simulink library "ConverterLibrary"  (R2026a)
settings: Solver=VariableStepAuto
undefined symbols (not defined in the file or in its folder): DiscIntNeverNeededParam, dspblkCoreblockFVToolHelper, gcbh, gridInverter
libraries: fl_lib x240, nesl_utility x221, ee_lib x208, slpidlib x28, eeGeneralControl x12, simulink x9, eeTransforms x4, simulink_extras x1, eePowerMeasurement x1
(part 7 of 30)

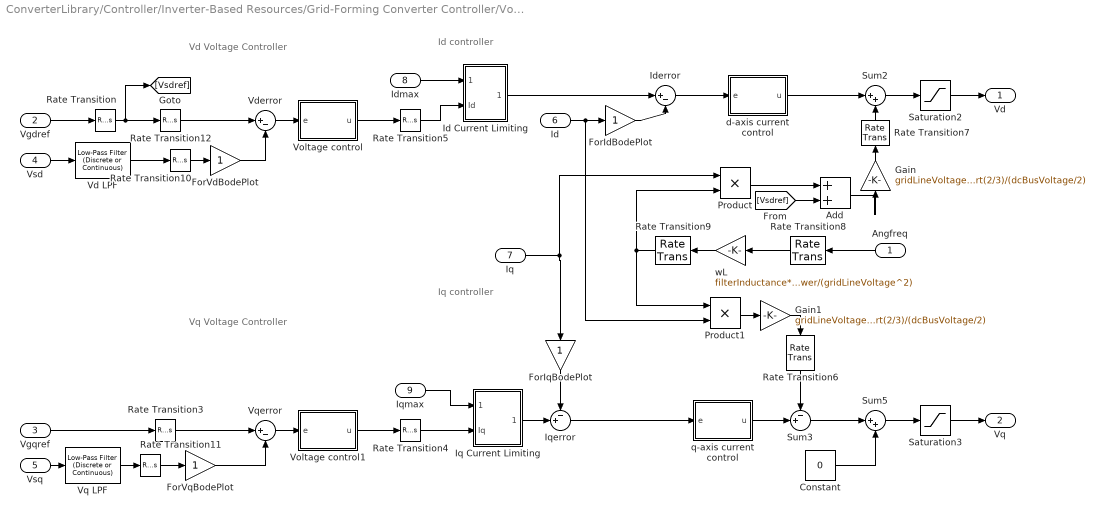
== system ConverterLibrary/Controller/Inverter-Based Resources/Grid-Forming Converter Controller/VoltageCurrentControl/Controller ==
  note: Vq Voltage Controller
  note: Iq controller
  note: Vd Voltage Controller
  note: Id controller
  Angfreq : Inport
  Vgdref : Inport  Port=2
  Vgqref : Inport  Port=3
  Vsd : Inport  Port=4
  Vsq : Inport  Port=5
  Id : Inport  Port=6
  Iq : Inport  Port=7
  Idmax : Inport  Port=8
  Iqmax : Inport  Port=9
  Add : Sum
  Constant : Constant  Value=0  SampleTime=currentControlTs
  ForIdBodePlot : Gain
  ForIqBodePlot : Gain
  ForVdBodePlot : Gain
  ForVqBodePlot : Gain
  Gain : Gain  Gain=gridLineVoltage*sqrt(2/3)/(dcBusVoltage/2)
  Gain1 : Gain  Gain=gridLineVoltage*sqrt(2/3)/(dcBusVoltage/2)
  Id Current Limiting : Subsystem
  Iderror : Sum  Inputs=|+-
  Iq Current Limiting : Subsystem
  Iqerror : Sum  Inputs=-+|
  Product : Product
  Product1 : Product
  Rate Transition{,3..12} (11 alike) : RateTransition
  Saturation2 : Saturate  UpperLimit=4  LowerLimit=-3
  Saturation3 : Saturate  UpperLimit=3  LowerLimit=-3
  Sum2 : Sum  Inputs=|++
  Sum3 : Sum  Inputs=-+|
  Sum5 : Sum  Inputs=|++
  Vd LPF : eeGeneralControl/Low-Pass Filter (Discrete or Continuous)  K=1  T=vdvqLPFTimeConst  B=inf  A=-inf  init_option=Specify as parameter  x0=0  Ts=voltControlTs
  Vderror : Sum  Inputs=|+-
  Voltage control : Subsystem
  Voltage control1 : Subsystem
  Vq LPF : eeGeneralControl/Low-Pass Filter (Discrete or Continuous)  K=1  T=vdvqLPFTimeConst  B=inf  A=-inf  init_option=Inherited from block input  x0=0  Ts=voltControlTs
  Vqerror : Sum  Inputs=|+-
  d-axis current control : Subsystem
  q-axis current control : Subsystem
  wL : Gain  Gain=filterInductance*power/(gridLineVoltage^2)
  Vd : Outport  VectorParamsAs1DForOutWhenUnconnected=off
  Vq : Outport  Port=2  VectorParamsAs1DForOutWhenUnconnected=off
  wires:
  Rate Transition12/1 -> Vderror/1
  Rate Transition11/1 -> ForVqBodePlot/1
  Rate Transition10/1 -> ForVdBodePlot/1
  Vd LPF/1 -> Rate Transition10/1
  ForVqBodePlot/1 -> Vqerror/2
  ForVdBodePlot/1 -> Vderror/2
  Rate Transition9/1 -> Product1/1, Product/2
  Vq LPF/1 -> Rate Transition11/1
  Rate Transition8/1 -> wL/1
  Rate Transition7/1 -> Sum2/2
  Rate Transition6/1 -> Sum3/1
  Rate Transition5/1 -> Id Current Limiting/2(Id)
  Rate Transition4/1 -> Iq Current Limiting/2(Iq)
  Rate Transition3/1 -> Vqerror/1
  Rate Transition/1 -> Rate Transition12/1, [Vsdref]
  Vgdref/1 -> Rate Transition/1
  Id Current Limiting/1(Idref) -> Iderror/1
  ForIqBodePlot/1 -> Iqerror/1
  ForIdBodePlot/1 -> Iderror/2
  Vsd/1 -> Vd LPF/1
  Voltage control1/1(u) -> Rate Transition4/1
  Iq Current Limiting/1(Iqref) -> Iqerror/2
  Idmax/1 -> Id Current Limiting/1(Imax)
  Voltage control/1(u) -> Rate Transition5/1
  Gain/1 -> Rate Transition7/1
  Add/1 -> Gain/1
  [Vsdref] -> Add/2
  Gain1/1 -> Rate Transition6/1
  Vqerror/1 -> Voltage control1/1(e)
  Vgqref/1 -> Rate Transition3/1
  Iqmax/1 -> Iq Current Limiting/1(Imax)
  Vderror/1 -> Voltage control/1(e)
  Id/1 -> ForIdBodePlot/1, Product1/2
  Vsq/1 -> Vq LPF/1
  Sum5/1 -> Saturation3/1
  Sum3/1 -> Sum5/1
  q-axis current control/1(u) -> Sum3/2
  Sum2/1 -> Saturation2/1
  d-axis current control/1(u) -> Sum2/1
  Product/1 -> Add/1
  Product1/1 -> Gain1/1
  Saturation2/1 -> Vd/1
  Saturation3/1 -> Vq/1
  Iderror/1 -> d-axis current control/1(e)
  Constant/1 -> Sum5/2
  Angfreq/1 -> Rate Transition8/1
  Iq/1 -> Product/1, ForIqBodePlot/1
  wL/1 -> Rate Transition9/1
  Iqerror/1 -> q-axis current control/1(e)

== system ConverterLibrary/Controller/Inverter-Based Resources/Grid-Forming Converter Controller/VoltageCurrentControl/Modulation Signal ==
  Vd : Inport
  Vq : Inport  Port=2
  Angle : Inport  Port=3
  Constant : Constant  Value=0
  Inverse Park Transform : eeTransforms/Inverse Park Transform  AxisAlignment=D-axis  PowerInvariant=off
  Mux1 : Mux  Inputs=3
  Saturation2 : Saturate  UpperLimit=1  LowerLimit=-1
  mabc : Outport  VectorParamsAs1DForOutWhenUnconnected=off
  wires:
  Vq/1 -> Mux1/2
  Angle/1 -> Inverse Park Transform/2
  Vd/1 -> Mux1/1
  Constant/1 -> Mux1/3
  Saturation2/1 -> mabc/1
  Mux1/1 -> Inverse Park Transform/1
  Inverse Park Transform/1 -> Saturation2/1

== system ConverterLibrary/Controller/Non-Isolated DC-DC Converters/Non-Isolated DC-DC Controller/Duty Feedforward/Feedforward Law ==
  voltageReferencePu : Inport
  inputVoltagePuOut : Inport  Port=2
  Boost : Subsystem  VariantControl=Boost
  Buck : Subsystem  VariantControl=Buck
  BuckBoost : Subsystem  VariantControl=BuckBoost
  dutyFeedforward : Outport

== system ConverterLibrary/Controller/Non-Isolated DC-DC Converters/Non-Isolated DC-DC Controller/Loop Structure/DoubleLoop ==
  voltageControllerOutput : Inport
  inductorCurrentPu : Inport  Port=2
  trimUpperLimit : Inport  Port=3
  trimLowerLimit : Inport  Port=4
  Current Controller : Subsystem  Variant=on  VariantControlMode=label  LabelModeActiveChoice=PIContinuous
  Sum : Sum  Inputs=|+-
  dutyTrim : Outport
  wires:
  Current Controller/1(vc) -> dutyTrim/1
  trimLowerLimit/1 -> Current Controller/3(lo)
  trimUpperLimit/1 -> Current Controller/2(up)
  Sum/1 -> Current Controller/1(error)
  inductorCurrentPu/1 -> Sum/2
  voltageControllerOutput/1 -> Sum/1

== system ConverterLibrary/Controller/Non-Isolated DC-DC Converters/Non-Isolated DC-DC Controller/Loop Structure/SingleLoop ==
  voltageControllerOutput : Inport
  inductorCurrentPu : Inport  Port=2
  trimUpperLimit : Inport  Port=3
  trimLowerLimit : Inport  Port=4
  Inductor Current Unused : Terminator
  Trim Clamp Lower : MinMax  Function=max  Inputs=2
  Trim Clamp Upper : MinMax  Inputs=2
  dutyTrim : Outport
  wires:
  Trim Clamp Lower/1 -> dutyTrim/1
  trimLowerLimit/1 -> Trim Clamp Lower/2
  Trim Clamp Upper/1 -> Trim Clamp Lower/1
  trimUpperLimit/1 -> Trim Clamp Upper/2
  voltageControllerOutput/1 -> Trim Clamp Upper/1
  inductorCurrentPu/1 -> Inductor Current Unused/1

== system ConverterLibrary/Controller/Non-Isolated DC-DC Converters/Non-Isolated DC-DC Controller/Output Mode/DutyCycle ==
  duty : Inport
  G : Outport
  wires:
  duty/1 -> G/1

== system ConverterLibrary/Controller/Non-Isolated DC-DC Converters/Non-Isolated DC-DC Controller/Output Mode/PWMSignal ==
  duty : Inport
  Gate Select : Selector  InputPortWidth=2  IndexOptions=Index vector (dialog)  Indices=gateIndices  OutputSizes=1
  Gate To Double : DataTypeConversion  OutDataTypeStr=double
  Half Bridge PWM Generator : Subsystem
  G : Outport
  wires:
  Gate Select/1 -> G/1
  Gate To Double/1 -> Gate Select/1
  Half Bridge PWM Generator/1(G) -> Gate To Double/1
  duty/1 -> Half Bridge PWM Generator/1(duty)

== system ConverterLibrary/Controller/Non-Isolated DC-DC Converters/Non-Isolated DC-DC Controller/Voltage Controller/PIContinuous ==
  error : Inport
  PI Controller : slpidlib/PID Controller  Controller=PI  Form=Parallel  TimeDomain=Continuous-time  UseExternalTs=off  SampleTime=-1  IntegratorMethod=Forward Euler  FilterMethod=Forward Euler  ControllerParametersSource=internal  P=KpVoltage  I=KiVoltage  UseKiTs=off  D=0  UseExternalDerivativeSource=off  N=100  UseFilter=on  TunerSelectOption=Transfer Function Based (PID Tuner App)  InitialConditionSource=internal  InitialConditionForIntegrator=voltageIntegratorInit  InitialConditionForFilter=0  DifferentiatorICPrevScaledInput=0  ExternalReset=none  TrackingMode=off  Kt=1  LimitOutput=on  SatLimitsSource=internal  UpperSaturationLimit=voltageLimitUpper  LowerSaturationLimit=voltageLimitLower  LinearizeAsGain=on  AntiWindupMode=clamping  Kb=1  LimitIntegrator=on  UpperIntegratorSaturationLimit=voltageLimitUpper  LowerIntegratorSaturationLimit=voltageLimitLower  POutMin=[]  POutMax=[]  IOutMin=[]  IOutMax=[]  DOutMin=[]  DOutMax=[]  NOutMin=[]  NOutMax=[]  SumOutMin=[]  SumOutMax=[]  SaturationOutMin=[]  SaturationOutMax=[]  PParamMin=[]  PParamMax=[]  IParamMin=[]  IParamMax=[]  DParamMin=[]  DParamMax=[]  NParamMin=[]  NParamMax=[]  KbParamMin=[]  KbParamMax=[]  KtParamMin=[]  KtParamMax=[]  KbOutMin=[]  KbOutMax=[]  KtOutMin=[]  KtOutMax=[]  IntegratorOutMin=[]  IntegratorOutMax=[]  FilterOutMin=[]  FilterOutMax=[]  SumI1OutMin=[]  SumI1OutMax=[]  SumI2OutMin=[]  SumI2OutMax=[]  SumI3OutMin=[]  SumI3OutMax=[]  SumI4OutMin=[]  SumI4OutMax=[]  SumDOutMin=[]  SumDOutMax=[]  DifferentiatorOutMin=[]  DifferentiatorOutMax=[]  FilterDiffOutCoefMin=[]  FilterDiffOutCoefMax=[]  ReciprocalOutMin=[]  ReciprocalOutMax=[]  SumDenOutMin=[]  SumDenOutMax=[]  SumNumOutMin=[]  SumNumOutMax=[]  DivideOutMin=[]  DivideOutMax=[]  UdiffTsProdOutMin=[]  UdiffTsProdOutMax=[]  NTsProdOutMin=[]  NTsProdOutMax=[]  UintegralTsProdOutMin=[]  UintegralTsProdOutMax=[]  UngainTsProdOutMin=[]  UngainTsProdOutMax=[]  ClampingZeroOutDataTypeStr=Inherit: Inherit via back propagation  ClampingZeroOutMin=[]  ClampingZeroOutMax=[]  FilterDenConstantOutDataTypeStr=Inherit: Inherit via back propagation  FilterDenConstantOutMin=[]  FilterDenConstantOutMax=[]  PCopyOutDataTypeStr=Inherit: Inherit via back propagation  PCopyOutMin=[]  PCopyOutMax=[]  NCopyOutDataTypeStr=Inherit: Inherit via back propagation  NCopyOutMin=[]  NCopyOutMax=[]  IntegratorContinuousStateAttributes=''  IntegratorStateMustResolveToSignalObject=off  IntegratorRTWStateStorageClass=Auto  FilterContinuousStateAttributes=''  FilterStateMustResolveToSignalObject=off  FilterRTWStateStorageClass=Auto  ParallelPVariant=InternalParameters  IdealPVariant=Disabled  IVariant=InternalParameters  DVariant=Disabled  IntegratorVariant=Continuous  SatVariant=Enabled  AWVariant=ContClampingParallel  PCopyVariant=Disabled  TRVariant=Disabled  FdbkBlocksVariant=Forward  IdealPFdbkVariant=Disabled  SatFdbkVariant=Disabled  DerivativeFilterVariant=Disabled  NVariant=Disabled  NCopyVariant=Disabled_SignalSpec  FilterICVariant=Disabled  IntegratorICVariant=InternalICs  ExternalResetVariant=Disabled  TRSumVariant=Passthrough  SumFdbkVariant=Disabled  SumVariant=Sum_PI  TsampFilterVariant=InternalTs  TsampNgainVariant=Passthrough  TsampIntegralVariant=Disabled_SignalSpec  ExternalSaturationOutDataTypeStr=Inherit: Same as second input  DerivativeSourceVariant=Disabled  PreIntVariant=InternalPreInt
  vc : Outport
  wires:
  PI Controller/1 -> vc/1
  error/1 -> PI Controller/1

== system ConverterLibrary/Controller/Non-Isolated DC-DC Converters/Non-Isolated DC-DC Controller/Voltage Controller/PIDiscrete ==
  error : Inport
  PI Controller : slpidlib/PID Controller  Controller=PI  Form=Parallel  TimeDomain=Discrete-time  UseExternalTs=off  SampleTime=TsVoltage  IntegratorMethod=Backward Euler  FilterMethod=Forward Euler  ControllerParametersSource=internal  P=KpVoltage  I=KiVoltage  UseKiTs=off  D=0  UseExternalDerivativeSource=off  N=100  UseFilter=on  TunerSelectOption=Transfer Function Based (PID Tuner App)  InitialConditionSource=internal  InitialConditionForIntegrator=voltageIntegratorInit  InitialConditionForFilter=0  DifferentiatorICPrevScaledInput=0  ExternalReset=none  TrackingMode=off  Kt=1  LimitOutput=on  SatLimitsSource=internal  UpperSaturationLimit=voltageLimitUpper  LowerSaturationLimit=voltageLimitLower  LinearizeAsGain=on  AntiWindupMode=clamping  Kb=1  LimitIntegrator=on  UpperIntegratorSaturationLimit=voltageLimitUpper  LowerIntegratorSaturationLimit=voltageLimitLower  POutMin=[]  POutMax=[]  IOutMin=[]  IOutMax=[]  DOutMin=[]  DOutMax=[]  NOutMin=[]  NOutMax=[]  SumOutMin=[]  SumOutMax=[]  SaturationOutMin=[]  SaturationOutMax=[]  PParamMin=[]  PParamMax=[]  IParamMin=[]  IParamMax=[]  DParamMin=[]  DParamMax=[]  NParamMin=[]  NParamMax=[]  KbParamMin=[]  KbParamMax=[]  KtParamMin=[]  KtParamMax=[]  KbOutMin=[]  KbOutMax=[]  KtOutMin=[]  KtOutMax=[]  IntegratorOutMin=[]  IntegratorOutMax=[]  FilterOutMin=[]  FilterOutMax=[]  SumI1OutMin=[]  SumI1OutMax=[]  SumI2OutMin=[]  SumI2OutMax=[]  SumI3OutMin=[]  SumI3OutMax=[]  SumI4OutMin=[]  SumI4OutMax=[]  SumDOutMin=[]  SumDOutMax=[]  DifferentiatorOutMin=[]  DifferentiatorOutMax=[]  FilterDiffOutCoefMin=[]  FilterDiffOutCoefMax=[]  ReciprocalOutMin=[]  ReciprocalOutMax=[]  SumDenOutMin=[]  SumDenOutMax=[]  SumNumOutMin=[]  SumNumOutMax=[]  DivideOutMin=[]  DivideOutMax=[]  UdiffTsProdOutMin=[]  UdiffTsProdOutMax=[]  NTsProdOutMin=[]  NTsProdOutMax=[]  UintegralTsProdOutMin=[]  UintegralTsProdOutMax=[]  UngainTsProdOutMin=[]  UngainTsProdOutMax=[]  ClampingZeroOutDataTypeStr=Inherit: Inherit via back propagation  ClampingZeroOutMin=[]  ClampingZeroOutMax=[]  FilterDenConstantOutDataTypeStr=Inherit: Inherit via back propagation  FilterDenConstantOutMin=[]  FilterDenConstantOutMax=[]  PCopyOutDataTypeStr=Inherit: Inherit via back propagation  PCopyOutMin=[]  PCopyOutMax=[]  NCopyOutDataTypeStr=Inherit: Inherit via back propagation  NCopyOutMin=[]  NCopyOutMax=[]  IntegratorContinuousStateAttributes=''  IntegratorStateMustResolveToSignalObject=off  IntegratorRTWStateStorageClass=Auto  FilterContinuousStateAttributes=''  FilterStateMustResolveToSignalObject=off  FilterRTWStateStorageClass=Auto  ParallelPVariant=InternalParameters  IdealPVariant=Disabled  IVariant=InternalParameters  DVariant=Disabled  IntegratorVariant=Discrete  SatVariant=Enabled  AWVariant=DiscClampingParallel  PCopyVariant=Disabled  TRVariant=Disabled  FdbkBlocksVariant=Feedback  IdealPFdbkVariant=Passthrough  SatFdbkVariant=Passthrough  DerivativeFilterVariant=Disabled  NVariant=Disabled  NCopyVariant=Disabled_SignalSpec  FilterICVariant=Disabled  IntegratorICVariant=InternalICs  ExternalResetVariant=Disabled  TRSumVariant=Passthrough  SumFdbkVariant=Enabled  SumVariant=Sum_PI  TsampFilterVariant=InternalTs  TsampNgainVariant=Passthrough  TsampIntegralVariant=Disabled_SignalSpec  ExternalSaturationOutDataTypeStr=Inherit: Same as second input  DerivativeSourceVariant=Disabled  PreIntVariant=InternalPreInt
  vc : Outport
  wires:
  PI Controller/1 -> vc/1
  error/1 -> PI Controller/1

== system ConverterLibrary/Controller/PWM Generators/CLLC PWM Generator/Primary Gate Signal/Leg Gate Logic ==
  Ton : Inport
  Toff : Inport  Port=2
  S : Inport  Port=3
  After Turn Off : RelationalOperator
  After Turn On : RelationalOperator
  Pulse Window : Logic  Operator=XOR
  To Double : DataTypeConversion  OutDataTypeStr=double
  gates : Outport
  wires:
  Ton/1 -> After Turn On/2
  Toff/1 -> After Turn Off/2
  S/1 -> After Turn Off/1, After Turn On/1
  After Turn On/1 -> Pulse Window/1
  After Turn Off/1 -> Pulse Window/2
  Pulse Window/1 -> To Double/1
  To Double/1 -> gates/1

== system ConverterLibrary/Controller/PWM Generators/CLLC PWM Generator/Primary Gate Signal/Ramp Mode ==
  Tsw : Inport
  FixedStep : Subsystem  VariantControl=FixedStep
  VariableStep : Subsystem  VariantControl=VariableStep
  S : Outport

== system ConverterLibrary/Controller/PWM Generators/CLLC PWM Generator/Synchronous Rectifier/Conduction Detect ==
  Isec : Inport
  Conduction Pair : Mux  Inputs=2
  Forward Conduction : RelationalOperator
  Forward Threshold : Constant  Value=Ith
  Rectifier Gate Map : Selector  InputPortWidth=2  IndexOptions=Index vector (dialog)  Indices=[1 2 2 1]  OutputSizes=1
  Reverse Conduction : RelationalOperator  Operator=<=
  Reverse Threshold : Constant  Value=-Ith
  permit : Outport
  wires:
  Isec/1 -> Forward Conduction/1, Reverse Conduction/1
  Forward Threshold/1 -> Forward Conduction/2
  Reverse Threshold/1 -> Reverse Conduction/2
  Forward Conduction/1 -> Conduction Pair/1
  Reverse Conduction/1 -> Conduction Pair/2
  Conduction Pair/1 -> Rectifier Gate Map/1
  Rectifier Gate Map/1 -> permit/1

== system ConverterLibrary/Controller/PWM Generators/CLLC PWM Generator/Synchronous Rectifier/Region Select ==
  primaryGates : Inport
  fpu : Inport  Port=2
  permit : Inport  Port=3
  Above Resonance : Subsystem
  Below Resonance : Subsystem
  If : If  IfExpression=u1 <= fpuSrLower  ElseIfExpressions=u1 >= fpuSrUpper  SampleTime=0
  Rectifier Gates : Merge  Inputs=3
  Within Band : Subsystem
  Gs : Outport
  wires:
  fpu/1 -> If/1
  If/1 -> Below Resonance/Action
  primaryGates/1 -> Below Resonance/1(primaryGates), Above Resonance/1(primaryGates), Within Band/1(primaryGates)
  permit/1 -> Below Resonance/2(permit), Above Resonance/2(permit), Within Band/2(permit)
  Below Resonance/1(Gs) -> Rectifier Gates/1
  If/2 -> Above Resonance/Action
  Above Resonance/1(Gs) -> Rectifier Gates/2
  If/3 -> Within Band/Action
  Within Band/1(Gs) -> Rectifier Gates/3
  Rectifier Gates/1 -> Gs/1

== system ConverterLibrary/Controller/PWM Generators/CLLC PWM Generator/Synchronous Rectifier/Turn On Delay ==
  condition : Inport
  Delay Elapsed : RelationalOperator
  Delay Time : Constant  Value=Tsr
  Logic To Double : DataTypeConversion  OutDataTypeStr=double
  Rate Offset : Bias  Bias=-1
  Rate Swing : Gain  Gain=2
  Rectifier Gate Window : Logic
  Rectifier Ramp Mode : Subsystem  Variant=on  VariantControlMode=label  LabelModeActiveChoice=VariableStep
  Gs : Outport
  wires:
  condition/1 -> Logic To Double/1, Rectifier Gate Window/1
  Logic To Double/1 -> Rate Swing/1
  Rate Swing/1 -> Rate Offset/1
  Rate Offset/1 -> Rectifier Ramp Mode/1(rate)
  Rectifier Ramp Mode/1(S) -> Delay Elapsed/1
  Delay Time/1 -> Delay Elapsed/2
  Delay Elapsed/1 -> Rectifier Gate Window/2
  Rectifier Gate Window/1 -> Gs/1

== system ConverterLibrary/Controller/PWM Generators/Complementary PWM Generator/Ramp Mode/FixedStep ==
  rate : Inport
  Dead Time Timer : DiscreteIntegrator  SampleTime=Ts  LimitOutput=on  UpperSaturationLimit=Tdead  LowerSaturationLimit=0  ICPrevOutput=DiscIntNeverNeededParam  ICPrevScaledInput=DiscIntNeverNeededParam
  S : Outport
  wires:
  rate/1 -> Dead Time Timer/1
  Dead Time Timer/1 -> S/1

== system ConverterLibrary/Controller/PWM Generators/Complementary PWM Generator/Ramp Mode/VariableStep ==
  rate : Inport
  Dead Time Timer : Integrator  LimitOutput=on  UpperSaturationLimit=Tdead  LowerSaturationLimit=0
  S : Outport
  wires:
  rate/1 -> Dead Time Timer/1
  Dead Time Timer/1 -> S/1

== system ConverterLibrary/Controller/PWM Generators/DAB PWM Generator/Ramp Mode/FixedStep ==
  Tsw : Inport
  Initial Ramp Value : InitialCondition  Value=0
  Overshoot Residual : Sum  Inputs=-+
  Period Reached : RelationalOperator  Operator=>  ZeroCross=off
  Time Ramp : DiscreteIntegrator  ExternalReset=rising  InitialConditionSource=external  SampleTime=Ts  ShowStatePort=on  ICPrevOutput=DiscIntNeverNeededParam  ICPrevScaledInput=DiscIntNeverNeededParam
  Unit Rate : Constant
  S : Outport
  wires:
  Unit Rate/1 -> Time Ramp/1
  Period Reached/1 -> Time Ramp/2
  Time Ramp/1 -> S/1
  Tsw/1 -> Overshoot Residual/1, Period Reached/2
  Time Ramp/State -> Period Reached/1, Overshoot Residual/2
  Overshoot Residual/1 -> Initial Ramp Value/1
  Initial Ramp Value/1 -> Time Ramp/3

== system ConverterLibrary/Controller/PWM Generators/DAB PWM Generator/Ramp Mode/VariableStep ==
  Tsw : Inport
  Initial Ramp Value : InitialCondition  Value=0
  Overshoot Residual : Sum  Inputs=-+
  Period Reached : RelationalOperator  Operator=>
  Time Ramp : Integrator  ExternalReset=rising  InitialConditionSource=external  ShowStatePort=on
  Unit Rate : Constant
  S : Outport
  wires:
  Unit Rate/1 -> Time Ramp/1
  Period Reached/1 -> Time Ramp/2
  Time Ramp/1 -> S/1
  Tsw/1 -> Overshoot Residual/1, Period Reached/2
  Time Ramp/State -> Period Reached/1, Overshoot Residual/2
  Overshoot Residual/1 -> Initial Ramp Value/1
  Initial Ramp Value/1 -> Time Ramp/3

== system ConverterLibrary/Controller/PWM Generators/Full Bridge PWM Generator/Ramp Mode/FixedStep ==
  Tsw : Inport
  Initial Ramp Value : InitialCondition  Value=0
  Overshoot Residual : Sum  Inputs=-+
  Period Reached : RelationalOperator  Operator=>  ZeroCross=off
  Time Ramp : DiscreteIntegrator  ExternalReset=rising  InitialConditionSource=external  SampleTime=Ts  ShowStatePort=on  ICPrevOutput=DiscIntNeverNeededParam  ICPrevScaledInput=DiscIntNeverNeededParam
  Unit Rate : Constant
  S : Outport
  wires:
  Unit Rate/1 -> Time Ramp/1
  Period Reached/1 -> Time Ramp/2
  Time Ramp/1 -> S/1
  Tsw/1 -> Overshoot Residual/1, Period Reached/2
  Time Ramp/State -> Period Reached/1, Overshoot Residual/2
  Overshoot Residual/1 -> Initial Ramp Value/1
  Initial Ramp Value/1 -> Time Ramp/3

== system ConverterLibrary/Controller/PWM Generators/Full Bridge PWM Generator/Ramp Mode/VariableStep ==
  Tsw : Inport
  Initial Ramp Value : InitialCondition  Value=0
  Overshoot Residual : Sum  Inputs=-+
  Period Reached : RelationalOperator  Operator=>
  Time Ramp : Integrator  ExternalReset=rising  InitialConditionSource=external  ShowStatePort=on
  Unit Rate : Constant
  S : Outport
  wires:
  Unit Rate/1 -> Time Ramp/1
  Period Reached/1 -> Time Ramp/2
  Time Ramp/1 -> S/1
  Tsw/1 -> Overshoot Residual/1, Period Reached/2
  Time Ramp/State -> Period Reached/1, Overshoot Residual/2
  Overshoot Residual/1 -> Initial Ramp Value/1
  Initial Ramp Value/1 -> Time Ramp/3

== system ConverterLibrary/Controller/PWM Generators/Half Bridge PWM Generator/Ramp Mode/FixedStep ==
  Tsw : Inport
  Initial Ramp Value : InitialCondition  Value=0
  Overshoot Residual : Sum  Inputs=-+
  Period Reached : RelationalOperator  Operator=>  ZeroCross=off
  Time Ramp : DiscreteIntegrator  ExternalReset=rising  InitialConditionSource=external  SampleTime=Ts  ShowStatePort=on  ICPrevOutput=DiscIntNeverNeededParam  ICPrevScaledInput=DiscIntNeverNeededParam
  Unit Rate : Constant
  S : Outport
  wires:
  Unit Rate/1 -> Time Ramp/1
  Period Reached/1 -> Time Ramp/2
  Time Ramp/1 -> S/1
  Tsw/1 -> Overshoot Residual/1, Period Reached/2
  Time Ramp/State -> Period Reached/1, Overshoot Residual/2
  Overshoot Residual/1 -> Initial Ramp Value/1
  Initial Ramp Value/1 -> Time Ramp/3

== system ConverterLibrary/Controller/PWM Generators/Half Bridge PWM Generator/Ramp Mode/VariableStep ==
  Tsw : Inport
  Initial Ramp Value : InitialCondition  Value=0
  Overshoot Residual : Sum  Inputs=-+
  Period Reached : RelationalOperator  Operator=>
  Time Ramp : Integrator  ExternalReset=rising  InitialConditionSource=external  ShowStatePort=on
  Unit Rate : Constant
  S : Outport
  wires:
  Unit Rate/1 -> Time Ramp/1
  Period Reached/1 -> Time Ramp/2
  Time Ramp/1 -> S/1
  Tsw/1 -> Overshoot Residual/1, Period Reached/2
  Time Ramp/State -> Period Reached/1, Overshoot Residual/2
  Overshoot Residual/1 -> Initial Ramp Value/1
  Initial Ramp Value/1 -> Time Ramp/3

== system ConverterLibrary/Controller/PWM Generators/LLC PWM Generator/Ramp Mode/FixedStep ==
  Tsw : Inport
  Initial Ramp Value : InitialCondition  Value=0
  Overshoot Residual : Sum  Inputs=-+
  Period Reached : RelationalOperator  Operator=>  ZeroCross=off
  Time Ramp : DiscreteIntegrator  ExternalReset=rising  InitialConditionSource=external  SampleTime=Ts  ShowStatePort=on  ICPrevOutput=DiscIntNeverNeededParam  ICPrevScaledInput=DiscIntNeverNeededParam
  Unit Rate : Constant
  S : Outport
  wires:
  Unit Rate/1 -> Time Ramp/1
  Period Reached/1 -> Time Ramp/2
  Time Ramp/1 -> S/1
  Tsw/1 -> Overshoot Residual/1, Period Reached/2
  Time Ramp/State -> Period Reached/1, Overshoot Residual/2
  Overshoot Residual/1 -> Initial Ramp Value/1
  Initial Ramp Value/1 -> Time Ramp/3

== system ConverterLibrary/Controller/PWM Generators/LLC PWM Generator/Ramp Mode/VariableStep ==
  Tsw : Inport
  Initial Ramp Value : InitialCondition  Value=0
  Overshoot Residual : Sum  Inputs=-+
  Period Reached : RelationalOperator  Operator=>
  Time Ramp : Integrator  ExternalReset=rising  InitialConditionSource=external  ShowStatePort=on
  Unit Rate : Constant
  S : Outport
  wires:
  Unit Rate/1 -> Time Ramp/1
  Period Reached/1 -> Time Ramp/2
  Time Ramp/1 -> S/1
  Tsw/1 -> Overshoot Residual/1, Period Reached/2
  Time Ramp/State -> Period Reached/1, Overshoot Residual/2
  Overshoot Residual/1 -> Initial Ramp Value/1
  Initial Ramp Value/1 -> Time Ramp/3

== system ConverterLibrary/Controller/Power Factor Correction Converters/Boost PFC Controller/Current Controller/PIContinuous ==
  error : Inport
  up : Inport  Port=2
  lo : Inport  Port=3
  PI Controller : slpidlib/PID Controller  Controller=PI  Form=Parallel  TimeDomain=Continuous-time  UseExternalTs=off  SampleTime=-1  IntegratorMethod=Forward Euler  FilterMethod=Forward Euler  ControllerParametersSource=internal  P=KpCurrent  I=KiCurrent  UseKiTs=off  D=0  UseExternalDerivativeSource=off  N=100  UseFilter=on  TunerSelectOption=Transfer Function Based (PID Tuner App)  InitialConditionSource=internal  InitialConditionForIntegrator=max(dutyMin - 1, min(0, dutyMax))  InitialConditionForFilter=0  DifferentiatorICPrevScaledInput=0  ExternalReset=none  TrackingMode=off  Kt=1  LimitOutput=on  SatLimitsSource=external  UpperSaturationLimit=inf  LowerSaturationLimit=-inf  LinearizeAsGain=on  AntiWindupMode=clamping  Kb=1  LimitIntegrator=on  UpperIntegratorSaturationLimit=dutyMax  LowerIntegratorSaturationLimit=dutyMin - 1  POutMin=[]  POutMax=[]  IOutMin=[]  IOutMax=[]  DOutMin=[]  DOutMax=[]  NOutMin=[]  NOutMax=[]  SumOutMin=[]  SumOutMax=[]  SaturationOutMin=[]  SaturationOutMax=[]  PParamMin=[]  PParamMax=[]  IParamMin=[]  IParamMax=[]  DParamMin=[]  DParamMax=[]  NParamMin=[]  NParamMax=[]  KbParamMin=[]  KbParamMax=[]  KtParamMin=[]  KtParamMax=[]  KbOutMin=[]  KbOutMax=[]  KtOutMin=[]  KtOutMax=[]  IntegratorOutMin=[]  IntegratorOutMax=[]  FilterOutMin=[]  FilterOutMax=[]  SumI1OutMin=[]  SumI1OutMax=[]  SumI2OutMin=[]  SumI2OutMax=[]  SumI3OutMin=[]  SumI3OutMax=[]  SumI4OutMin=[]  SumI4OutMax=[]  SumDOutMin=[]  SumDOutMax=[]  DifferentiatorOutMin=[]  DifferentiatorOutMax=[]  FilterDiffOutCoefMin=[]  FilterDiffOutCoefMax=[]  ReciprocalOutMin=[]  ReciprocalOutMax=[]  SumDenOutMin=[]  SumDenOutMax=[]  SumNumOutMin=[]  SumNumOutMax=[]  DivideOutMin=[]  DivideOutMax=[]  UdiffTsProdOutMin=[]  UdiffTsProdOutMax=[]  NTsProdOutMin=[]  NTsProdOutMax=[]  UintegralTsProdOutMin=[]  UintegralTsProdOutMax=[]  UngainTsProdOutMin=[]  UngainTsProdOutMax=[]  ClampingZeroOutDataTypeStr=Inherit: Inherit via back propagation  ClampingZeroOutMin=[]  ClampingZeroOutMax=[]  FilterDenConstantOutDataTypeStr=Inherit: Inherit via back propagation  FilterDenConstantOutMin=[]  FilterDenConstantOutMax=[]  PCopyOutDataTypeStr=Inherit: Inherit via back propagation  PCopyOutMin=[]  PCopyOutMax=[]  NCopyOutDataTypeStr=Inherit: Inherit via back propagation  NCopyOutMin=[]  NCopyOutMax=[]  IntegratorContinuousStateAttributes=''  IntegratorStateMustResolveToSignalObject=off  IntegratorRTWStateStorageClass=Auto  FilterContinuousStateAttributes=''  FilterStateMustResolveToSignalObject=off  FilterRTWStateStorageClass=Auto  ParallelPVariant=InternalParameters  IdealPVariant=Disabled  IVariant=InternalParameters  DVariant=Disabled  IntegratorVariant=Continuous  SatVariant=External  AWVariant=ContClampingParallel  PCopyVariant=Disabled  TRVariant=Disabled  FdbkBlocksVariant=Forward  IdealPFdbkVariant=Disabled  SatFdbkVariant=Disabled  DerivativeFilterVariant=Disabled  NVariant=Disabled  NCopyVariant=Disabled_SignalSpec  FilterICVariant=Disabled  IntegratorICVariant=InternalICs  ExternalResetVariant=Disabled  TRSumVariant=Passthrough  SumFdbkVariant=Disabled  SumVariant=Sum_PI  TsampFilterVariant=InternalTs  TsampNgainVariant=Passthrough  TsampIntegralVariant=Disabled_SignalSpec  ExternalSaturationOutDataTypeStr=Inherit: Same as second input  DerivativeSourceVariant=Disabled  PreIntVariant=InternalPreInt
  vc : Outport
  wires:
  PI Controller/1 -> vc/1
  lo/1 -> PI Controller/3
  up/1 -> PI Controller/2
  error/1 -> PI Controller/1

== system ConverterLibrary/Controller/Power Factor Correction Converters/Boost PFC Controller/Current Controller/PIDiscrete ==
  error : Inport
  up : Inport  Port=2
  lo : Inport  Port=3
  PI Controller : slpidlib/PID Controller  Controller=PI  Form=Parallel  TimeDomain=Discrete-time  UseExternalTs=off  SampleTime=TsCurrent  IntegratorMethod=Backward Euler  FilterMethod=Forward Euler  ControllerParametersSource=internal  P=KpCurrent  I=KiCurrent  UseKiTs=off  D=0  UseExternalDerivativeSource=off  N=100  UseFilter=on  TunerSelectOption=Transfer Function Based (PID Tuner App)  InitialConditionSource=internal  InitialConditionForIntegrator=max(dutyMin - 1, min(0, dutyMax))  InitialConditionForFilter=0  DifferentiatorICPrevScaledInput=0  ExternalReset=none  TrackingMode=off  Kt=1  LimitOutput=on  SatLimitsSource=external  UpperSaturationLimit=inf  LowerSaturationLimit=-inf  LinearizeAsGain=on  AntiWindupMode=clamping  Kb=1  LimitIntegrator=on  UpperIntegratorSaturationLimit=dutyMax  LowerIntegratorSaturationLimit=dutyMin - 1  POutMin=[]  POutMax=[]  IOutMin=[]  IOutMax=[]  DOutMin=[]  DOutMax=[]  NOutMin=[]  NOutMax=[]  SumOutMin=[]  SumOutMax=[]  SaturationOutMin=[]  SaturationOutMax=[]  PParamMin=[]  PParamMax=[]  IParamMin=[]  IParamMax=[]  DParamMin=[]  DParamMax=[]  NParamMin=[]  NParamMax=[]  KbParamMin=[]  KbParamMax=[]  KtParamMin=[]  KtParamMax=[]  KbOutMin=[]  KbOutMax=[]  KtOutMin=[]  KtOutMax=[]  IntegratorOutMin=[]  IntegratorOutMax=[]  FilterOutMin=[]  FilterOutMax=[]  SumI1OutMin=[]  SumI1OutMax=[]  SumI2OutMin=[]  SumI2OutMax=[]  SumI3OutMin=[]  SumI3OutMax=[]  SumI4OutMin=[]  SumI4OutMax=[]  SumDOutMin=[]  SumDOutMax=[]  DifferentiatorOutMin=[]  DifferentiatorOutMax=[]  FilterDiffOutCoefMin=[]  FilterDiffOutCoefMax=[]  ReciprocalOutMin=[]  ReciprocalOutMax=[]  SumDenOutMin=[]  SumDenOutMax=[]  SumNumOutMin=[]  SumNumOutMax=[]  DivideOutMin=[]  DivideOutMax=[]  UdiffTsProdOutMin=[]  UdiffTsProdOutMax=[]  NTsProdOutMin=[]  NTsProdOutMax=[]  UintegralTsProdOutMin=[]  UintegralTsProdOutMax=[]  UngainTsProdOutMin=[]  UngainTsProdOutMax=[]  ClampingZeroOutDataTypeStr=Inherit: Inherit via back propagation  ClampingZeroOutMin=[]  ClampingZeroOutMax=[]  FilterDenConstantOutDataTypeStr=Inherit: Inherit via back propagation  FilterDenConstantOutMin=[]  FilterDenConstantOutMax=[]  PCopyOutDataTypeStr=Inherit: Inherit via back propagation  PCopyOutMin=[]  PCopyOutMax=[]  NCopyOutDataTypeStr=Inherit: Inherit via back propagation  NCopyOutMin=[]  NCopyOutMax=[]  IntegratorContinuousStateAttributes=''  IntegratorStateMustResolveToSignalObject=off  IntegratorRTWStateStorageClass=Auto  FilterContinuousStateAttributes=''  FilterStateMustResolveToSignalObject=off  FilterRTWStateStorageClass=Auto  ParallelPVariant=InternalParameters  IdealPVariant=Disabled  IVariant=InternalParameters  DVariant=Disabled  IntegratorVariant=Discrete  SatVariant=External  AWVariant=DiscClampingParallel  PCopyVariant=Disabled  TRVariant=Disabled  FdbkBlocksVariant=Feedback  IdealPFdbkVariant=Passthrough  SatFdbkVariant=Passthrough  DerivativeFilterVariant=Disabled  NVariant=Disabled  NCopyVariant=Disabled_SignalSpec  FilterICVariant=Disabled  IntegratorICVariant=InternalICs  ExternalResetVariant=Disabled  TRSumVariant=Passthrough  SumFdbkVariant=Enabled  SumVariant=Sum_PI  TsampFilterVariant=InternalTs  TsampNgainVariant=Passthrough  TsampIntegralVariant=Disabled_SignalSpec  ExternalSaturationOutDataTypeStr=Inherit: Same as second input  DerivativeSourceVariant=Disabled  PreIntVariant=InternalPreInt
  vc : Outport
  wires:
  PI Controller/1 -> vc/1
  lo/1 -> PI Controller/3
  up/1 -> PI Controller/2
  error/1 -> PI Controller/1

== system ConverterLibrary/Controller/Power Factor Correction Converters/Boost PFC Controller/Output Mode/DutyCycle ==
  duty : Inport
  G : Outport
  wires:
  duty/1 -> G/1

== system ConverterLibrary/Controller/Power Factor Correction Converters/Boost PFC Controller/Output Mode/PWMSignal ==
  duty : Inport
  Gate Drive : Subsystem
  Leg Gate Logic : Subsystem
  Pulse Time : Gain  Gain=1/Fsw
  Pulse Width Limit : Saturate  UpperLimit=dutyMax  LowerLimit=dutyMin
  Ramp Mode : Subsystem  Variant=on  VariantControlMode=label  LabelModeActiveChoice=VariableStep
  Switching Period : Constant  Value=1/Fsw
  Turn On Time : Constant  Value=dutyMin/Fsw
  G : Outport
  wires:
  Gate Drive/1(gateVoltage) -> G/1
  Leg Gate Logic/1(gates) -> Gate Drive/1(gateLogic)
  Ramp Mode/1(S) -> Leg Gate Logic/3(S)
  Switching Period/1 -> Ramp Mode/1(Tsw)
  Turn On Time/1 -> Leg Gate Logic/1(Ton)
  Pulse Time/1 -> Leg Gate Logic/2(Toff)
  Pulse Width Limit/1 -> Pulse Time/1
  duty/1 -> Pulse Width Limit/1

== system ConverterLibrary/Controller/Power Factor Correction Converters/Boost PFC Controller/Voltage Controller/PIContinuous ==
  error : Inport
  PI Controller : slpidlib/PID Controller  Controller=PI  Form=Parallel  TimeDomain=Continuous-time  UseExternalTs=off  SampleTime=-1  IntegratorMethod=Forward Euler  FilterMethod=Forward Euler  ControllerParametersSource=internal  P=KpVoltage  I=KiVoltage  UseKiTs=off  D=0  UseExternalDerivativeSource=off  N=100  UseFilter=on  TunerSelectOption=Transfer Function Based (PID Tuner App)  InitialConditionSource=internal  InitialConditionForIntegrator=max(-PrefPu, min(0, max(0, iRefPeakMaxPu - PrefPu)))  InitialConditionForFilter=0  DifferentiatorICPrevScaledInput=0  ExternalReset=none  TrackingMode=off  Kt=1  LimitOutput=on  SatLimitsSource=internal  UpperSaturationLimit=max(0, iRefPeakMaxPu - PrefPu)  LowerSaturationLimit=-PrefPu  LinearizeAsGain=on  AntiWindupMode=clamping  Kb=1  LimitIntegrator=on  UpperIntegratorSaturationLimit=max(0, iRefPeakMaxPu - PrefPu)  LowerIntegratorSaturationLimit=-PrefPu  POutMin=[]  POutMax=[]  IOutMin=[]  IOutMax=[]  DOutMin=[]  DOutMax=[]  NOutMin=[]  NOutMax=[]  SumOutMin=[]  SumOutMax=[]  SaturationOutMin=[]  SaturationOutMax=[]  PParamMin=[]  PParamMax=[]  IParamMin=[]  IParamMax=[]  DParamMin=[]  DParamMax=[]  NParamMin=[]  NParamMax=[]  KbParamMin=[]  KbParamMax=[]  KtParamMin=[]  KtParamMax=[]  KbOutMin=[]  KbOutMax=[]  KtOutMin=[]  KtOutMax=[]  IntegratorOutMin=[]  IntegratorOutMax=[]  FilterOutMin=[]  FilterOutMax=[]  SumI1OutMin=[]  SumI1OutMax=[]  SumI2OutMin=[]  SumI2OutMax=[]  SumI3OutMin=[]  SumI3OutMax=[]  SumI4OutMin=[]  SumI4OutMax=[]  SumDOutMin=[]  SumDOutMax=[]  DifferentiatorOutMin=[]  DifferentiatorOutMax=[]  FilterDiffOutCoefMin=[]  FilterDiffOutCoefMax=[]  ReciprocalOutMin=[]  ReciprocalOutMax=[]  SumDenOutMin=[]  SumDenOutMax=[]  SumNumOutMin=[]  SumNumOutMax=[]  DivideOutMin=[]  DivideOutMax=[]  UdiffTsProdOutMin=[]  UdiffTsProdOutMax=[]  NTsProdOutMin=[]  NTsProdOutMax=[]  UintegralTsProdOutMin=[]  UintegralTsProdOutMax=[]  UngainTsProdOutMin=[]  UngainTsProdOutMax=[]  ClampingZeroOutDataTypeStr=Inherit: Inherit via back propagation  ClampingZeroOutMin=[]  ClampingZeroOutMax=[]  FilterDenConstantOutDataTypeStr=Inherit: Inherit via back propagation  FilterDenConstantOutMin=[]  FilterDenConstantOutMax=[]  PCopyOutDataTypeStr=Inherit: Inherit via back propagation  PCopyOutMin=[]  PCopyOutMax=[]  NCopyOutDataTypeStr=Inherit: Inherit via back propagation  NCopyOutMin=[]  NCopyOutMax=[]  IntegratorContinuousStateAttributes=''  IntegratorStateMustResolveToSignalObject=off  IntegratorRTWStateStorageClass=Auto  FilterContinuousStateAttributes=''  FilterStateMustResolveToSignalObject=off  FilterRTWStateStorageClass=Auto  ParallelPVariant=InternalParameters  IdealPVariant=Disabled  IVariant=InternalParameters  DVariant=Disabled  IntegratorVariant=Continuous  SatVariant=Enabled  AWVariant=ContClampingParallel  PCopyVariant=Disabled  TRVariant=Disabled  FdbkBlocksVariant=Forward  IdealPFdbkVariant=Disabled  SatFdbkVariant=Disabled  DerivativeFilterVariant=Disabled  NVariant=Disabled  NCopyVariant=Disabled_SignalSpec  FilterICVariant=Disabled  IntegratorICVariant=InternalICs  ExternalResetVariant=Disabled  TRSumVariant=Passthrough  SumFdbkVariant=Disabled  SumVariant=Sum_PI  TsampFilterVariant=InternalTs  TsampNgainVariant=Passthrough  TsampIntegralVariant=Disabled_SignalSpec  ExternalSaturationOutDataTypeStr=Inherit: Same as second input  DerivativeSourceVariant=Disabled  PreIntVariant=InternalPreInt
  vc : Outport
  wires:
  PI Controller/1 -> vc/1
  error/1 -> PI Controller/1

== system ConverterLibrary/Controller/Power Factor Correction Converters/Boost PFC Controller/Voltage Controller/PIDiscrete ==
  error : Inport
  PI Controller : slpidlib/PID Controller  Controller=PI  Form=Parallel  TimeDomain=Discrete-time  UseExternalTs=off  SampleTime=TsVoltage  IntegratorMethod=Backward Euler  FilterMethod=Forward Euler  ControllerParametersSource=internal  P=KpVoltage  I=KiVoltage  UseKiTs=off  D=0  UseExternalDerivativeSource=off  N=100  UseFilter=on  TunerSelectOption=Transfer Function Based (PID Tuner App)  InitialConditionSource=internal  InitialConditionForIntegrator=max(-PrefPu, min(0, max(0, iRefPeakMaxPu - PrefPu)))  InitialConditionForFilter=0  DifferentiatorICPrevScaledInput=0  ExternalReset=none  TrackingMode=off  Kt=1  LimitOutput=on  SatLimitsSource=internal  UpperSaturationLimit=max(0, iRefPeakMaxPu - PrefPu)  LowerSaturationLimit=-PrefPu  LinearizeAsGain=on  AntiWindupMode=clamping  Kb=1  LimitIntegrator=on  UpperIntegratorSaturationLimit=max(0, iRefPeakMaxPu - PrefPu)  LowerIntegratorSaturationLimit=-PrefPu  POutMin=[]  POutMax=[]  IOutMin=[]  IOutMax=[]  DOutMin=[]  DOutMax=[]  NOutMin=[]  NOutMax=[]  SumOutMin=[]  SumOutMax=[]  SaturationOutMin=[]  SaturationOutMax=[]  PParamMin=[]  PParamMax=[]  IParamMin=[]  IParamMax=[]  DParamMin=[]  DParamMax=[]  NParamMin=[]  NParamMax=[]  KbParamMin=[]  KbParamMax=[]  KtParamMin=[]  KtParamMax=[]  KbOutMin=[]  KbOutMax=[]  KtOutMin=[]  KtOutMax=[]  IntegratorOutMin=[]  IntegratorOutMax=[]  FilterOutMin=[]  FilterOutMax=[]  SumI1OutMin=[]  SumI1OutMax=[]  SumI2OutMin=[]  SumI2OutMax=[]  SumI3OutMin=[]  SumI3OutMax=[]  SumI4OutMin=[]  SumI4OutMax=[]  SumDOutMin=[]  SumDOutMax=[]  DifferentiatorOutMin=[]  DifferentiatorOutMax=[]  FilterDiffOutCoefMin=[]  FilterDiffOutCoefMax=[]  ReciprocalOutMin=[]  ReciprocalOutMax=[]  SumDenOutMin=[]  SumDenOutMax=[]  SumNumOutMin=[]  SumNumOutMax=[]  DivideOutMin=[]  DivideOutMax=[]  UdiffTsProdOutMin=[]  UdiffTsProdOutMax=[]  NTsProdOutMin=[]  NTsProdOutMax=[]  UintegralTsProdOutMin=[]  UintegralTsProdOutMax=[]  UngainTsProdOutMin=[]  UngainTsProdOutMax=[]  ClampingZeroOutDataTypeStr=Inherit: Inherit via back propagation  ClampingZeroOutMin=[]  ClampingZeroOutMax=[]  FilterDenConstantOutDataTypeStr=Inherit: Inherit via back propagation  FilterDenConstantOutMin=[]  FilterDenConstantOutMax=[]  PCopyOutDataTypeStr=Inherit: Inherit via back propagation  PCopyOutMin=[]  PCopyOutMax=[]  NCopyOutDataTypeStr=Inherit: Inherit via back propagation  NCopyOutMin=[]  NCopyOutMax=[]  IntegratorContinuousStateAttributes=''  IntegratorStateMustResolveToSignalObject=off  IntegratorRTWStateStorageClass=Auto  FilterContinuousStateAttributes=''  FilterStateMustResolveToSignalObject=off  FilterRTWStateStorageClass=Auto  ParallelPVariant=InternalParameters  IdealPVariant=Disabled  IVariant=InternalParameters  DVariant=Disabled  IntegratorVariant=Discrete  SatVariant=Enabled  AWVariant=DiscClampingParallel  PCopyVariant=Disabled  TRVariant=Disabled  FdbkBlocksVariant=Feedback  IdealPFdbkVariant=Passthrough  SatFdbkVariant=Passthrough  DerivativeFilterVariant=Disabled  NVariant=Disabled  NCopyVariant=Disabled_SignalSpec  FilterICVariant=Disabled  IntegratorICVariant=InternalICs  ExternalResetVariant=Disabled  TRSumVariant=Passthrough  SumFdbkVariant=Enabled  SumVariant=Sum_PI  TsampFilterVariant=InternalTs  TsampNgainVariant=Passthrough  TsampIntegralVariant=Disabled_SignalSpec  ExternalSaturationOutDataTypeStr=Inherit: Same as second input  DerivativeSourceVariant=Disabled  PreIntVariant=InternalPreInt
  vc : Outport
  wires:
  PI Controller/1 -> vc/1
  error/1 -> PI Controller/1

== system ConverterLibrary/Controller/Power Factor Correction Converters/Interleaved Boost PFC Controller/Current Balance/Balance Controller ==
  error : Inport
  PIContinuous : Subsystem  VariantControl=PIContinuous
  PIDiscrete : Subsystem  VariantControl=PIDiscrete
  vc : Outport

== system ConverterLibrary/Controller/Power Factor Correction Converters/Interleaved Boost PFC Controller/Current Controller/PIContinuous ==
  error : Inport
  up : Inport  Port=2
  lo : Inport  Port=3
  PI Controller : slpidlib/PID Controller  Controller=PI  Form=Parallel  TimeDomain=Continuous-time  UseExternalTs=off  SampleTime=-1  IntegratorMethod=Forward Euler  FilterMethod=Forward Euler  ControllerParametersSource=internal  P=KpCurrent  I=KiCurrent  UseKiTs=off  D=0  UseExternalDerivativeSource=off  N=100  UseFilter=on  TunerSelectOption=Transfer Function Based (PID Tuner App)  InitialConditionSource=internal  InitialConditionForIntegrator=max(dutyMin - 1, min(0, dutyMax))  InitialConditionForFilter=0  DifferentiatorICPrevScaledInput=0  ExternalReset=none  TrackingMode=off  Kt=1  LimitOutput=on  SatLimitsSource=external  UpperSaturationLimit=inf  LowerSaturationLimit=-inf  LinearizeAsGain=on  AntiWindupMode=clamping  Kb=1  LimitIntegrator=on  UpperIntegratorSaturationLimit=dutyMax  LowerIntegratorSaturationLimit=dutyMin - 1  POutMin=[]  POutMax=[]  IOutMin=[]  IOutMax=[]  DOutMin=[]  DOutMax=[]  NOutMin=[]  NOutMax=[]  SumOutMin=[]  SumOutMax=[]  SaturationOutMin=[]  SaturationOutMax=[]  PParamMin=[]  PParamMax=[]  IParamMin=[]  IParamMax=[]  DParamMin=[]  DParamMax=[]  NParamMin=[]  NParamMax=[]  KbParamMin=[]  KbParamMax=[]  KtParamMin=[]  KtParamMax=[]  KbOutMin=[]  KbOutMax=[]  KtOutMin=[]  KtOutMax=[]  IntegratorOutMin=[]  IntegratorOutMax=[]  FilterOutMin=[]  FilterOutMax=[]  SumI1OutMin=[]  SumI1OutMax=[]  SumI2OutMin=[]  SumI2OutMax=[]  SumI3OutMin=[]  SumI3OutMax=[]  SumI4OutMin=[]  SumI4OutMax=[]  SumDOutMin=[]  SumDOutMax=[]  DifferentiatorOutMin=[]  DifferentiatorOutMax=[]  FilterDiffOutCoefMin=[]  FilterDiffOutCoefMax=[]  ReciprocalOutMin=[]  ReciprocalOutMax=[]  SumDenOutMin=[]  SumDenOutMax=[]  SumNumOutMin=[]  SumNumOutMax=[]  DivideOutMin=[]  DivideOutMax=[]  UdiffTsProdOutMin=[]  UdiffTsProdOutMax=[]  NTsProdOutMin=[]  NTsProdOutMax=[]  UintegralTsProdOutMin=[]  UintegralTsProdOutMax=[]  UngainTsProdOutMin=[]  UngainTsProdOutMax=[]  ClampingZeroOutDataTypeStr=Inherit: Inherit via back propagation  ClampingZeroOutMin=[]  ClampingZeroOutMax=[]  FilterDenConstantOutDataTypeStr=Inherit: Inherit via back propagation  FilterDenConstantOutMin=[]  FilterDenConstantOutMax=[]  PCopyOutDataTypeStr=Inherit: Inherit via back propagation  PCopyOutMin=[]  PCopyOutMax=[]  NCopyOutDataTypeStr=Inherit: Inherit via back propagation  NCopyOutMin=[]  NCopyOutMax=[]  IntegratorContinuousStateAttributes=''  IntegratorStateMustResolveToSignalObject=off  IntegratorRTWStateStorageClass=Auto  FilterContinuousStateAttributes=''  FilterStateMustResolveToSignalObject=off  FilterRTWStateStorageClass=Auto  ParallelPVariant=InternalParameters  IdealPVariant=Disabled  IVariant=InternalParameters  DVariant=Disabled  IntegratorVariant=Continuous  SatVariant=External  AWVariant=ContClampingParallel  PCopyVariant=Disabled  TRVariant=Disabled  FdbkBlocksVariant=Forward  IdealPFdbkVariant=Disabled  SatFdbkVariant=Disabled  DerivativeFilterVariant=Disabled  NVariant=Disabled  NCopyVariant=Disabled_SignalSpec  FilterICVariant=Disabled  IntegratorICVariant=InternalICs  ExternalResetVariant=Disabled  TRSumVariant=Passthrough  SumFdbkVariant=Disabled  SumVariant=Sum_PI  TsampFilterVariant=InternalTs  TsampNgainVariant=Passthrough  TsampIntegralVariant=Disabled_SignalSpec  ExternalSaturationOutDataTypeStr=Inherit: Same as second input  DerivativeSourceVariant=Disabled  PreIntVariant=InternalPreInt
  vc : Outport
  wires:
  PI Controller/1 -> vc/1
  lo/1 -> PI Controller/3
  up/1 -> PI Controller/2
  error/1 -> PI Controller/1

== system ConverterLibrary/Controller/Power Factor Correction Converters/Interleaved Boost PFC Controller/Current Controller/PIDiscrete ==
  error : Inport
  up : Inport  Port=2
  lo : Inport  Port=3
  PI Controller : slpidlib/PID Controller  Controller=PI  Form=Parallel  TimeDomain=Discrete-time  UseExternalTs=off  SampleTime=TsCurrent  IntegratorMethod=Backward Euler  FilterMethod=Forward Euler  ControllerParametersSource=internal  P=KpCurrent  I=KiCurrent  UseKiTs=off  D=0  UseExternalDerivativeSource=off  N=100  UseFilter=on  TunerSelectOption=Transfer Function Based (PID Tuner App)  InitialConditionSource=internal  InitialConditionForIntegrator=max(dutyMin - 1, min(0, dutyMax))  InitialConditionForFilter=0  DifferentiatorICPrevScaledInput=0  ExternalReset=none  TrackingMode=off  Kt=1  LimitOutput=on  SatLimitsSource=external  UpperSaturationLimit=inf  LowerSaturationLimit=-inf  LinearizeAsGain=on  AntiWindupMode=clamping  Kb=1  LimitIntegrator=on  UpperIntegratorSaturationLimit=dutyMax  LowerIntegratorSaturationLimit=dutyMin - 1  POutMin=[]  POutMax=[]  IOutMin=[]  IOutMax=[]  DOutMin=[]  DOutMax=[]  NOutMin=[]  NOutMax=[]  SumOutMin=[]  SumOutMax=[]  SaturationOutMin=[]  SaturationOutMax=[]  PParamMin=[]  PParamMax=[]  IParamMin=[]  IParamMax=[]  DParamMin=[]  DParamMax=[]  NParamMin=[]  NParamMax=[]  KbParamMin=[]  KbParamMax=[]  KtParamMin=[]  KtParamMax=[]  KbOutMin=[]  KbOutMax=[]  KtOutMin=[]  KtOutMax=[]  IntegratorOutMin=[]  IntegratorOutMax=[]  FilterOutMin=[]  FilterOutMax=[]  SumI1OutMin=[]  SumI1OutMax=[]  SumI2OutMin=[]  SumI2OutMax=[]  SumI3OutMin=[]  SumI3OutMax=[]  SumI4OutMin=[]  SumI4OutMax=[]  SumDOutMin=[]  SumDOutMax=[]  DifferentiatorOutMin=[]  DifferentiatorOutMax=[]  FilterDiffOutCoefMin=[]  FilterDiffOutCoefMax=[]  ReciprocalOutMin=[]  ReciprocalOutMax=[]  SumDenOutMin=[]  SumDenOutMax=[]  SumNumOutMin=[]  SumNumOutMax=[]  DivideOutMin=[]  DivideOutMax=[]  UdiffTsProdOutMin=[]  UdiffTsProdOutMax=[]  NTsProdOutMin=[]  NTsProdOutMax=[]  UintegralTsProdOutMin=[]  UintegralTsProdOutMax=[]  UngainTsProdOutMin=[]  UngainTsProdOutMax=[]  ClampingZeroOutDataTypeStr=Inherit: Inherit via back propagation  ClampingZeroOutMin=[]  ClampingZeroOutMax=[]  FilterDenConstantOutDataTypeStr=Inherit: Inherit via back propagation  FilterDenConstantOutMin=[]  FilterDenConstantOutMax=[]  PCopyOutDataTypeStr=Inherit: Inherit via back propagation  PCopyOutMin=[]  PCopyOutMax=[]  NCopyOutDataTypeStr=Inherit: Inherit via back propagation  NCopyOutMin=[]  NCopyOutMax=[]  IntegratorContinuousStateAttributes=''  IntegratorStateMustResolveToSignalObject=off  IntegratorRTWStateStorageClass=Auto  FilterContinuousStateAttributes=''  FilterStateMustResolveToSignalObject=off  FilterRTWStateStorageClass=Auto  ParallelPVariant=InternalParameters  IdealPVariant=Disabled  IVariant=InternalParameters  DVariant=Disabled  IntegratorVariant=Discrete  SatVariant=External  AWVariant=DiscClampingParallel  PCopyVariant=Disabled  TRVariant=Disabled  FdbkBlocksVariant=Feedback  IdealPFdbkVariant=Passthrough  SatFdbkVariant=Passthrough  DerivativeFilterVariant=Disabled  NVariant=Disabled  NCopyVariant=Disabled_SignalSpec  FilterICVariant=Disabled  IntegratorICVariant=InternalICs  ExternalResetVariant=Disabled  TRSumVariant=Passthrough  SumFdbkVariant=Enabled  SumVariant=Sum_PI  TsampFilterVariant=InternalTs  TsampNgainVariant=Passthrough  TsampIntegralVariant=Disabled_SignalSpec  ExternalSaturationOutDataTypeStr=Inherit: Same as second input  DerivativeSourceVariant=Disabled  PreIntVariant=InternalPreInt
  vc : Outport
  wires:
  PI Controller/1 -> vc/1
  lo/1 -> PI Controller/3
  up/1 -> PI Controller/2
  error/1 -> PI Controller/1

== system ConverterLibrary/Controller/Power Factor Correction Converters/Interleaved Boost PFC Controller/Output Mode/DutyCycle ==
  duty : Inport
  G : Outport
  wires:
  duty/1 -> G/1

== system ConverterLibrary/Controller/Power Factor Correction Converters/Interleaved Boost PFC Controller/Output Mode/PWMSignal ==
  duty : Inport
  Gate Drive : Subsystem
  Leg 2 Carrier Shift : Constant  Value=1/(Fsw*numberOfLegs)
  Leg 2 Shifted Time : Sum
  Leg 2 Wrap To Period : Math  Operator=mod
  Leg Carriers : Mux  Inputs=2
  Leg Gate Logic : Subsystem
  Pulse Time : Gain  Gain=1/Fsw
  Pulse Width Limit : Saturate  UpperLimit=dutyMax  LowerLimit=dutyMin
  Ramp Mode : Subsystem  Variant=on  VariantControlMode=label  LabelModeActiveChoice=VariableStep
  Switching Period : Constant  Value=1/Fsw
  Turn On Time : Constant  Value=dutyMin/Fsw
  G : Outport
  wires:
  duty/1 -> Pulse Width Limit/1
  Gate Drive/1(gateVoltage) -> G/1
  Leg Gate Logic/1(gates) -> Gate Drive/1(gateLogic)
  Leg Carriers/1 -> Leg Gate Logic/3(S)
  Leg 2 Wrap To Period/1 -> Leg Carriers/2
  Leg 2 Shifted Time/1 -> Leg 2 Wrap To Period/1
  Leg 2 Carrier Shift/1 -> Leg 2 Shifted Time/2
  Ramp Mode/1(S) -> Leg 2 Shifted Time/1, Leg Carriers/1
  Switching Period/1 -> Ramp Mode/1(Tsw), Leg 2 Wrap To Period/2
  Turn On Time/1 -> Leg Gate Logic/1(Ton)
  Pulse Time/1 -> Leg Gate Logic/2(Toff)
  Pulse Width Limit/1 -> Pulse Time/1
